simulink model "twiddle_coeff_1_test"  (Simulink 7.2)
settings: Solver=VariableStepDiscrete  StartTime=0.0  StopTime=1000  RelTol=1e-3
libraries: xbsIndex_r4 x15, casper_library_misc x3, simulink x1
settings Model: Creator=User  LastModifiedBy=root
settings OptimizationCC: InitFltsAndDblsToZero=on
settings DebuggingCC: SaveWithDisabledLinksMsg=none  SaveWithParameterizedLinksMsg=none

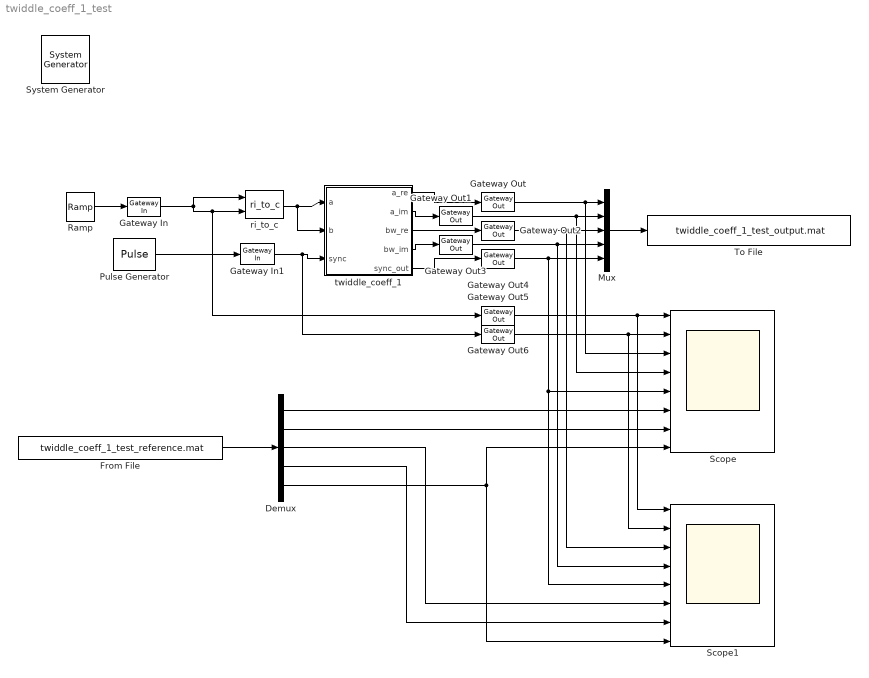
== system twiddle_coeff_1_test ==
  " System Generator" : xbsIndex_r4/ System Generator  Tag=genX  SystemSampleTime=-1  xilinxfamily=Virtex4  part=xc4vsx35  speed=-10  package=ff668  synthesis_tool=XST  clock_wrapper=Clock Enables  directory=./netlist  testbench=off  simulink_period=1  sysclk_period=100  dcm_input_clock_period=100  incr_netlist=off  trim_vbits=Everywhere in SubSystem  dbl_ovrd=According to Block Masks  core_generation=According to Block Masks  run_coregen=off  deprecated_control=off  eval_field=0  block_type=sysgen
      settings: block_version=10.1.1
  Demux : Demux  Outputs=5
  From File : FromFile  FileName=twiddle_coeff_1_test_reference.mat  SampleTime=1
  Gateway In : xbsIndex_r4/Gateway In  arith_type="Signed  (2's comp)"  n_bits=5  bin_pt=4  quantization=Truncate  overflow=Wrap  period=1  dbl_ovrd=off  timing_constraint=None  locs_specified=off  LOCs={}  hdl_port=on  block_type=gatewayin
      settings: infoedit="Gateway in block.  Converts inputs of type Simulink integer, double and fixed point to  Xilinx fixed point type.<P><P>Hardware notes:  In hardware these blocks become top level input ports."  block_version=10.1.1
  Gateway In1 : xbsIndex_r4/Gateway In  arith_type=Boolean  n_bits=16  bin_pt=14  quantization="Round  (unbiased: +/- Inf)"  overflow=Saturate  period=1  dbl_ovrd=off  timing_constraint=None  locs_specified=off  LOCs={}  hdl_port=on  block_type=gatewayin
      settings: infoedit="Gateway in block.  Converts inputs of type Simulink integer, double and fixed point to  Xilinx fixed point type.<P><P>Hardware notes:  In hardware these blocks become top level input ports."  block_version=10.1.1
  Gateway Out{,1..6} (7 alike) : xbsIndex_r4/Gateway Out  hdl_port=on  timing_constraint=None  locs_specified=off  LOCs={}  block_type=gatewayout
      settings: infoedit="Gateway out block.  Converts Xilinx fixed point inputs into ouputs of type Simulink integer, double, or fixed point.<P><P>Hardware notes:  In hardware these blocks become top level output ports or are discarded, depending on how they are configured."  block_version=10.1.1
  Mux : Mux  Inputs=5
  Pulse Generator : DiscretePulseGenerator  Period=256  PhaseDelay=7
  Ramp : simulink/Sources/Ramp  SystemSampleTime=-1  slope=1/2^5  start=0  X0=0
  Scope : Scope  NumInputPorts=8
      settings: TimeRange=1000  YMin=-1~0~-1~-1~0~-1~-1~-1  YMax=1~1~1~1~1~1~1~1
  Scope1 : Scope  NumInputPorts=8
      settings: YMin=-1~-1~-1~-1~-1~-1~-1~-1  YMax=1~1~1~1~1~1~1~1
  To File : ToFile  Filename=twiddle_coeff_1_test_output.mat  MatrixName=output
  ri_to_c : casper_library_misc/ri_to_c  SystemSampleTime=-1
  twiddle_coeff_1 : Subsystem  AncestorBlock=casper_library_ffts_twiddle/twiddle_coeff_1  mask(twiddle_coeff_1){FFTSize=5, input_bit_width=5, add_latency=2, mult_latency=3, bram_latency=2, conv_latency=1, opt_target=logic}
      mask prompts: FFTSize "FFT Size (2^?)"; input_bit_width "Input Bit Width"; add_latency "Add Latency"; mult_latency "Mult Latency"; bram_latency "BRAM Latency"; conv_latency "Convert latency"; opt_target "Use less"
      mask help:
      | Used in FFT library. Used when result of
      | coeff*(a+jb)=b-ja
      mask init:
      | set_param(gcb,'LinkStatus','inactive');
      | if(strcmp(opt_target, 'logic')), 
      |     latency = 'mult_latency+add_latency+bram_latency+conv_latency';
      | else,
      |     latency = 'mult_latency+add_latency*2+bram_latency+conv_latency';
      | end
      | set_param([gcb,'/delay0'], 'latency', latency);
      | set_param([gcb,'/delay1'], 'latency', latency);
      | set_param([gcb,'/delay2'], 'latency', latency);
      | set_param([gcb,'/delay3'], 'latency', latency);
      | set_param([gcb,'/negate'], 'latency', latency);
      mask StyleString: edit,edit,edit,edit,edit,edit,popup(logic|multipliers)
  wires:
  Ramp/1 -> Gateway In/1
  Pulse Generator/1 -> Gateway In1/1
  Gateway In1/1 -> Gateway Out6/1, twiddle_coeff_1/3(sync)
  Gateway Out/1 -> Mux/1, Scope/3
  Gateway Out1/1 -> Mux/2, Scope/4
  Gateway Out2/1 -> Mux/3, Scope1/3
  Gateway Out3/1 -> Mux/4, Scope1/4
  Gateway Out4/1 -> Mux/5, Scope/5, Scope1/5
  Mux/1 -> To File/1
  Gateway Out5/1 -> Scope/1, Scope1/1
  Gateway Out6/1 -> Scope/2, Scope1/2
  Gateway In/1 -> ri_to_c/1, ri_to_c/2, Gateway Out5/1
  ri_to_c/1 -> twiddle_coeff_1/2(b), twiddle_coeff_1/1(a)
  Demux/2 -> Scope/7
  Demux/5 -> Scope/8, Scope1/8
  Demux/1 -> Scope/6
  Demux/3 -> Scope1/6
  Demux/4 -> Scope1/7
  From File/1 -> Demux/1
  twiddle_coeff_1/1(a_re) -> Gateway Out/1
  twiddle_coeff_1/2(a_im) -> Gateway Out1/1
  twiddle_coeff_1/3(bw_re) -> Gateway Out2/1
  twiddle_coeff_1/4(bw_im) -> Gateway Out3/1
  twiddle_coeff_1/5(sync_out) -> Gateway Out4/1

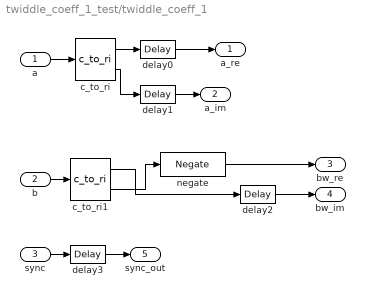
== system twiddle_coeff_1_test/twiddle_coeff_1 ==
  a : Inport  OutDataType=sfix(16)  OutScaling=2^0
  b : Inport  Port=2  OutDataType=sfix(16)  OutScaling=2^0
  sync : Inport  Port=3  OutDataType=sfix(16)  OutScaling=2^0
  c_to_ri : casper_library_misc/c_to_ri  SystemSampleTime=-1  n_bits=input_bit_width  bin_pt=input_bit_width-1
      settings: AttributesFormatString=5_4 r/i
  c_to_ri1 : casper_library_misc/c_to_ri  SystemSampleTime=-1  n_bits=input_bit_width  bin_pt=input_bit_width-1
      settings: AttributesFormatString=5_4 r/i
  delay{0..3} (4 alike) : xbsIndex_r4/Delay  en=off  latency=mult_latency+add_latency+bram_latency+conv_latency  dbl_ovrd=off  reg_retiming=on  block_type=delay
      settings: xl_area=[0, 0, 0, 0, 0, 0, 0]  block_version=9.1.01
  negate : xbsIndex_r4/Negate  precision=User Defined  arith_type="Signed  (2's comp)"  n_bits=input_bit_width  bin_pt=input_bit_width-1  quantization=Truncate  overflow=Wrap  en=off  latency=mult_latency+add_latency+bram_latency+conv_latency  dbl_ovrd=off  block_type=negate
      settings: xl_area=[0, 0, 0, 0, 0, 0, 0]  block_version=9.1.01
  a_re : Outport  OutDataType=sfix(16)  OutScaling=2^0
  a_im : Outport  Port=2  OutDataType=sfix(16)  OutScaling=2^0
  bw_re : Outport  Port=3  OutDataType=sfix(16)  OutScaling=2^0
  bw_im : Outport  Port=4  OutDataType=sfix(16)  OutScaling=2^0
  sync_out : Outport  Port=5  OutDataType=sfix(16)  OutScaling=2^0
  wires:
  c_to_ri/2 -> delay1/1
  c_to_ri/1 -> delay0/1
  b/1 -> c_to_ri1/1
  delay3/1 -> sync_out/1
  sync/1 -> delay3/1
  a/1 -> c_to_ri/1
  c_to_ri1/1 -> delay2/1
  negate/1 -> bw_re/1
  c_to_ri1/2 -> negate/1
  delay2/1 -> bw_im/1
  delay0/1 -> a_re/1
  delay1/1 -> a_im/1
